simulink model "FMT_RigidBodyRHS"  (R2026b)
settings: Solver=FixedStepDiscrete  StopTime=2  FixedStep=0.0005
settings Model: DataDictionary=Flight_Parameters.sldd  Creator=26718  LastModifiedBy=26718

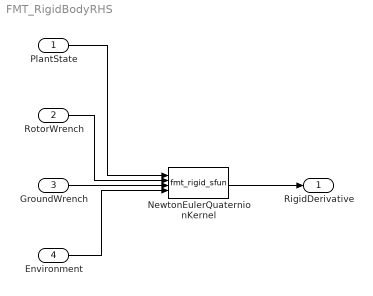
== system FMT_RigidBodyRHS ==
  PlantState : Inport  OutDataTypeStr=double  PortDimensions=17
  RotorWrench : Inport  Port=2  OutDataTypeStr=double  PortDimensions=6
  GroundWrench : Inport  Port=3  OutDataTypeStr=double  PortDimensions=6
  Environment : Inport  Port=4  OutDataTypeStr=double  PortDimensions=15
  NewtonEulerQuaternionKernel : S-Function  FunctionName=fmt_rigid_sfun  Parameters=PlantParameters  SFunctionDeploymentMode=off  EnableBusSupport=off
  RigidDerivative : Outport
  wires:
  NewtonEulerQuaternionKernel/1 -> RigidDerivative/1
  Environment/1 -> NewtonEulerQuaternionKernel/4
  GroundWrench/1 -> NewtonEulerQuaternionKernel/3
  RotorWrench/1 -> NewtonEulerQuaternionKernel/2
  PlantState/1 -> NewtonEulerQuaternionKernel/1
